simulink library "conventional_airplane_single_engine_lib"  (R2018b)
settings: Solver=VariableStepAuto  StartTime=0.0  StopTime=10.0  RelTol=1e-3
undefined symbols (not defined in the file or in its folder): airplane
libraries: actuators_lib x5, conventional_airplane_aerodynamics_lib x1, ground_lib x1, propulsion_lib x1, rigidBody_lib x1, flight_parameters_lib x1
settings Model: Creator=Ybeyer  LastModifiedBy=fabian
settings SFSimCC: SimUseLocalCustomCode=off
settings RTWCC: RTWUseLocalCustomCode=off
settings CodeAppCC: StateflowObjectComments=on

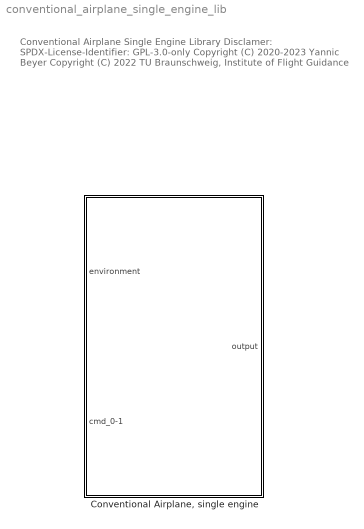
== system conventional_airplane_single_engine_lib ==
  note: Conventional Airplane Single Engine Library
      |
      | Disclamer:
      | SPDX-License-Identifier: GPL-3.0-only
      |
      | Copyright (C) 2020-2023 Yannic Beyer
      | Copyright (C) 2022 TU Braunschweig, Institute of Flight Guidance
  "Conventional Airplane, single engine" : Subsystem  mask{airplane=airplane}
      mask prompts: airplane "airplane struct"
      mask DialogControl DescGroupVar Prompt: Conventional Airplane, singe engine
      mask DialogControl DescTextVar Prompt: See conventionalAirplaneLoadParams for more information about the parameter struct.

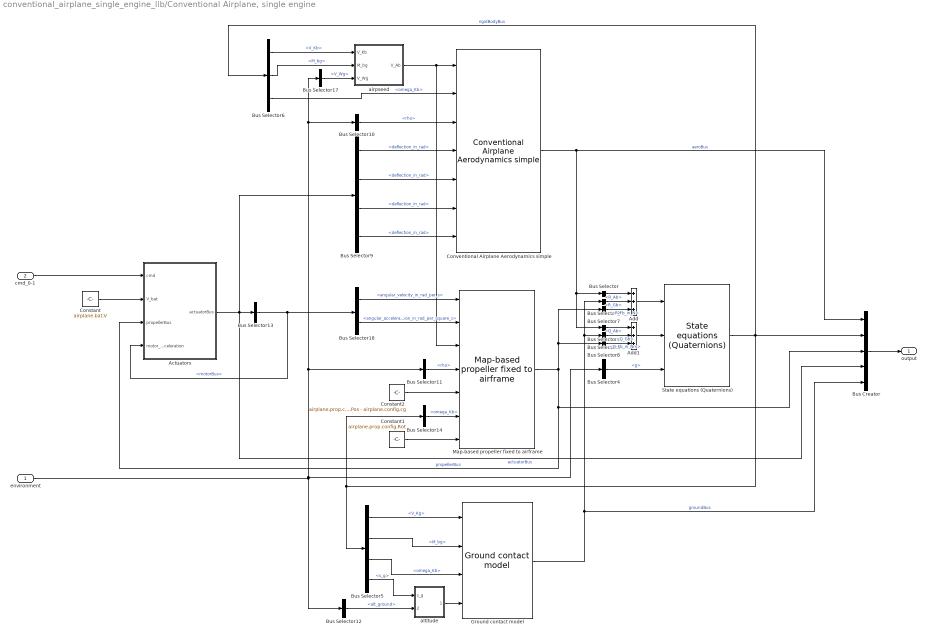
== system conventional_airplane_single_engine_lib/Conventional Airplane, single engine ==
  environment : Inport  OutDataTypeStr=Bus: envirBus
  cmd_0-1 : Inport  Port=2  OutDataTypeStr=Bus: cmdBus
  Actuators : Subsystem
  Add : Sum  Inputs=+++
  Add1 : Sum  Inputs=+++
  Bus Creator : BusCreator  Inputs=5
  Bus Selector : BusSelector  OutputSignals=R_Ab
  Bus Selector1 : BusSelector  OutputSignals=Q_Ab
  Bus Selector10 : BusSelector  OutputSignals=atmosphere.rho
  Bus Selector11 : BusSelector  OutputSignals=atmosphere.rho
  Bus Selector12 : BusSelector  OutputSignals=alt_ground
  Bus Selector13 : BusSelector  OutputSignals=motorBus
  Bus Selector14 : BusSelector  OutputSignals=omega_Kb
  Bus Selector17 : BusSelector  OutputSignals=wind.V_Wg
  Bus Selector18 : BusSelector  OutputSignals=angular_velocity_in_rad_per_s,angular_acceleration_in_rad_per_square_s
  Bus Selector2 : BusSelector  OutputSignals=forces_and_moments.R_Gb
  Bus Selector3 : BusSelector  OutputSignals=forces_and_moments.Q_Gb
  Bus Selector4 : BusSelector  OutputSignals=g
  Bus Selector5 : BusSelector  OutputSignals=V_Kg,M_bg,omega_Kb,s_g
  Bus Selector6 : BusSelector  OutputSignals=V_Kb,M_bg,omega_Kb
  Bus Selector7 : BusSelector  OutputSignals=R_Fb_in_N
  Bus Selector8 : BusSelector  OutputSignals=Q_Fb_in_Nm
  Bus Selector9 : BusSelector  OutputSignals=aileronsBus.deflection_in_rad,elevatorBus.deflection_in_rad,rudderBus.deflection_in_rad,htpTrimBus.deflection_in_rad
  Constant : Constant  Value=airplane.bat.V
  Constant1 : Constant  Value=airplane.prop.config.Rot
  Constant2 : Constant  Value=airplane.prop.config.Pos - airplane.config.cg
  Conventional Airplane Aerodynamics simple : conventional_airplane_aerodynamics_lib/Conventional Airplane Aerodynamics simple  aeroStruct=airplane.aero  xyz_cg_c=airplane.config.cg
      settings: SourceProductName=LADAC
  Ground contact model : ground_lib/Ground contact model  m=airplane.body.m  a_max=airplane.grnd.acc_max  xyz_c_hit=airplane.config.hitPoints  xyz_c_cg=airplane.config.cg  ground_softness_param=airplane.grnd.softness_parameter  k_h=airplane.grnd.spring_stiffness  k_dot_h=airplane.grnd.damping  mu=airplane.grnd.friction_coef  k_V=airplane.grnd.low_speed_friction_reduction_factor
      settings: SourceProductName=LADAC
  Map-based propeller fixed to airframe : propulsion_lib/Map-based propeller fixed to airframe  prop_map_fit=airplane.prop.map_fit  I_prop=airplane.prop.I  rotation_orientation=airplane.prop.dir
      settings: SourceProductName=LADAC
  State equations (Quaternions) : rigidBody_lib/State equations (Quaternions)  m=airplane.body.m  I=airplane.body.I  is_g_checked=on  g=10  omega_Kb_0=airplane.ic.omega_Kb  q_bg_0=airplane.ic.q_bg  V_Kb_0=airplane.ic.V_Kb  s_g_0=airplane.ic.s_Kg
      settings: SourceProductName=LADAC
  airpseed : Subsystem
  altitude : Subsystem
  output : Outport
  wires:
  Conventional Airplane Aerodynamics simple/1 -> Bus Selector1/1, Bus Selector/1, Bus Creator/1  "aeroBus"
  Bus Selector/1 -> Add/1  "<R_Ab>"
  Add/1 -> State equations (Quaternions)/1
  Add1/1 -> State equations (Quaternions)/2
  Bus Selector1/1 -> Add1/1  "<Q_Ab>"
  Bus Selector2/1 -> Add/2  "<R_Gb>"
  Ground contact model/1 -> Bus Creator/5, Bus Selector2/1, Bus Selector3/1  "groundBus"
  Bus Selector3/1 -> Add1/2  "<Q_Gb>"
  Bus Selector4/1 -> State equations (Quaternions)/3  "<g>"
  environment/1 -> Bus Selector11/1, Bus Selector17/1, Bus Selector10/1, Bus Selector4/1, Bus Selector12/1
  State equations (Quaternions)/1 -> Bus Selector6/1, Bus Creator/2, Bus Selector14/1, Bus Selector5/1  "rigidBodyBus"
  Bus Selector5/3 -> Ground contact model/3  "<omega_Kb>"
  Bus Selector5/2 -> Ground contact model/2  "<M_bg>"
  Bus Selector5/1 -> Ground contact model/1  "<V_Kg>"
  Bus Selector6/3 -> Conventional Airplane Aerodynamics simple/2  "<omega_Kb>"
  Bus Selector7/1 -> Add/3  "<R_Fb_in_N>"
  Map-based propeller fixed to airframe/1 -> Actuators/3(propellerBus), Bus Creator/3, Bus Selector8/1, Bus Selector7/1  "propellerBus"
  Bus Selector8/1 -> Add1/3  "<Q_Fb_in_Nm>"
  cmd_0-1/1 -> Actuators/1(cmd)
  Bus Selector9/1 -> Conventional Airplane Aerodynamics simple/4  "<deflection_in_rad>"
  Bus Selector9/2 -> Conventional Airplane Aerodynamics simple/5  "<deflection_in_rad>"
  Bus Selector9/3 -> Conventional Airplane Aerodynamics simple/6  "<deflection_in_rad>"
  Bus Selector9/4 -> Conventional Airplane Aerodynamics simple/7  "<deflection_in_rad>"
  Bus Selector10/1 -> Conventional Airplane Aerodynamics simple/3  "<rho>"
  Bus Selector11/1 -> Map-based propeller fixed to airframe/4  "<rho>"
  Bus Selector12/1 -> altitude/2(h_ground)  "<alt_ground>"
  altitude/1(alt_cg) -> Ground contact model/4
  Bus Selector14/1 -> Map-based propeller fixed to airframe/6  "<omega_Kb>"
  Bus Selector5/4 -> altitude/1(s_g)  "<s_g>"
  airpseed/1(V_Ab) -> Map-based propeller fixed to airframe/3, Conventional Airplane Aerodynamics simple/1
  Bus Selector6/1 -> airpseed/1(V_Kb)  "<V_Kb>"
  Bus Selector6/2 -> airpseed/2(M_bg)  "<M_bg>"
  Bus Selector17/1 -> airpseed/3(V_Wg)  "<V_Wg>"
  Bus Creator/1 -> output/1
  Constant1/1 -> Map-based propeller fixed to airframe/7
  Constant2/1 -> Map-based propeller fixed to airframe/5
  Bus Selector18/1 -> Map-based propeller fixed to airframe/1  "<angular_velocity_in_rad_per_s>"
  Bus Selector18/2 -> Map-based propeller fixed to airframe/2  "<angular_acceleration_in_rad_per_square_s>"
  Bus Selector13/1 -> Actuators/4(motor_acceleration), Bus Selector18/1  "<motorBus>"
  Constant/1 -> Actuators/2(V_bat)
  Actuators/1(actuatorBus) -> Bus Selector9/1, Bus Creator/4, Bus Selector13/1  "actuatorBus"

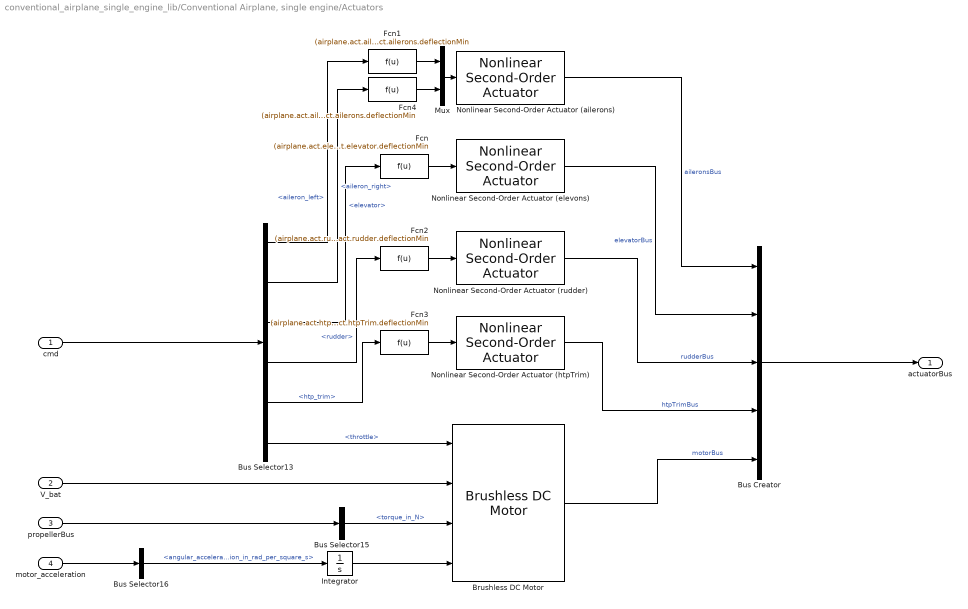
== system conventional_airplane_single_engine_lib/Conventional Airplane, single engine/Actuators ==
  cmd : Inport
  V_bat : Inport  Port=2
  propellerBus : Inport  Port=3
  motor_acceleration : Inport  Port=4
  Brushless DC Motor : actuators_lib/Brushless DC Motor  K_T=airplane.motor.KT  J_prop=airplane.prop.I  R_i=airplane.motor.R  IC_omega=0  omega_max=Inf  omega_min=0
      settings: SourceProductName=LADAC
  Bus Creator : BusCreator  Inputs=5
  Bus Selector13 : BusSelector  OutputSignals=aileron_left,aileron_right,elevator,rudder,htp_trim,throttle
  Bus Selector15 : BusSelector  OutputSignals=torque_in_N
  Bus Selector16 : BusSelector  OutputSignals=angular_acceleration_in_rad_per_square_s
  Fcn : Fcn  Expr=(airplane.act.elevator.deflectionMax - airplane.act.elevator.deflectionMin)*u + airplane.act.elevator.deflectionMin
  Fcn1 : Fcn  Expr=(airplane.act.ailerons.deflectionMax - airplane.act.ailerons.deflectionMin)*u + airplane.act.ailerons.deflectionMin
  Fcn2 : Fcn  Expr=(airplane.act.rudder.deflectionMax - airplane.act.rudder.deflectionMin)*u + airplane.act.rudder.deflectionMin
  Fcn3 : Fcn  Expr=(airplane.act.htpTrim.deflectionMax - airplane.act.htpTrim.deflectionMin)*u + airplane.act.htpTrim.deflectionMin
  Fcn4 : Fcn  Expr=(airplane.act.ailerons.deflectionMax - airplane.act.ailerons.deflectionMin)*u + airplane.act.ailerons.deflectionMin
  Integrator : Integrator  InitialCondition=airplane.ic.motor_speed  ContinuousStateAttributes='motor_speed'
  Mux : Mux  Inputs=2
  Nonlinear Second-Order Actuator (ailerons) : actuators_lib/Nonlinear Second-Order Actuator  omega=airplane.act.ailerons.naturalFrequency  d=airplane.act.ailerons.dampingRatio  A_max=airplane.act.ailerons.deflectionMax  A_min=airplane.act.ailerons.deflectionMin  dot_A_max=airplane.act.ailerons.deflectionRateMax  dot_A_min=-airplane.act.ailerons.deflectionRateMax  A_0=0  dot_A_0=0
      settings: SourceProductName=LADAC
  Nonlinear Second-Order Actuator (elevons) : actuators_lib/Nonlinear Second-Order Actuator  omega=airplane.act.elevator.naturalFrequency  d=airplane.act.elevator.dampingRatio  A_max=airplane.act.elevator.deflectionMax  A_min=airplane.act.elevator.deflectionMin  dot_A_max=airplane.act.elevator.deflectionRateMax  dot_A_min=-airplane.act.elevator.deflectionRateMax  A_0=0  dot_A_0=0
      settings: SourceProductName=LADAC
  Nonlinear Second-Order Actuator (htpTrim) : actuators_lib/Nonlinear Second-Order Actuator  omega=airplane.act.htpTrim.naturalFrequency  d=airplane.act.htpTrim.dampingRatio  A_max=airplane.act.htpTrim.deflectionMax  A_min=airplane.act.htpTrim.deflectionMin  dot_A_max=airplane.act.htpTrim.deflectionRateMax  dot_A_min=-airplane.act.htpTrim.deflectionRateMax  A_0=0  dot_A_0=0
      settings: SourceProductName=LADAC
  Nonlinear Second-Order Actuator (rudder) : actuators_lib/Nonlinear Second-Order Actuator  omega=airplane.act.rudder.naturalFrequency  d=airplane.act.rudder.dampingRatio  A_max=airplane.act.rudder.deflectionMax  A_min=airplane.act.rudder.deflectionMin  dot_A_max=airplane.act.rudder.deflectionRateMax  dot_A_min=-airplane.act.rudder.deflectionRateMax  A_0=0  dot_A_0=0
      settings: SourceProductName=LADAC
  actuatorBus : Outport
  wires:
  Bus Selector13/6 -> Brushless DC Motor/1  "<throttle>"
  Bus Selector16/1 -> Integrator/1  "<angular_acceleration_in_rad_per_square_s>"
  Bus Selector15/1 -> Brushless DC Motor/3  "<torque_in_N>"
  motor_acceleration/1 -> Bus Selector16/1
  Integrator/1 -> Brushless DC Motor/4
  Brushless DC Motor/1 -> Bus Creator/5  "motorBus"
  cmd/1 -> Bus Selector13/1
  V_bat/1 -> Brushless DC Motor/2
  propellerBus/1 -> Bus Selector15/1
  Bus Creator/1 -> actuatorBus/1
  Nonlinear Second-Order Actuator (rudder)/1 -> Bus Creator/3  "rudderBus"
  Nonlinear Second-Order Actuator (elevons)/1 -> Bus Creator/2  "elevatorBus"
  Nonlinear Second-Order Actuator (ailerons)/1 -> Bus Creator/1  "aileronsBus"
  Bus Selector13/1 -> Fcn1/1  "<aileron_left>"
  Bus Selector13/3 -> Fcn/1  "<elevator>"
  Bus Selector13/4 -> Fcn2/1  "<rudder>"
  Bus Selector13/2 -> Fcn4/1  "<aileron_right>"
  Bus Selector13/5 -> Fcn3/1  "<htp_trim>"
  Nonlinear Second-Order Actuator (htpTrim)/1 -> Bus Creator/4  "htpTrimBus"
  Fcn/1 -> Nonlinear Second-Order Actuator (elevons)/1
  Mux/1 -> Nonlinear Second-Order Actuator (ailerons)/1
  Fcn2/1 -> Nonlinear Second-Order Actuator (rudder)/1
  Fcn3/1 -> Nonlinear Second-Order Actuator (htpTrim)/1
  Fcn1/1 -> Mux/1
  Fcn4/1 -> Mux/2

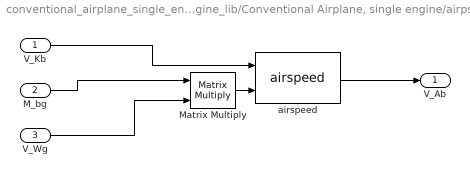
== system conventional_airplane_single_engine_lib/Conventional Airplane, single engine/airpseed ==
  V_Kb : Inport
  M_bg : Inport  Port=2
  V_Wg : Inport  Port=3
  Matrix Multiply : Product  Multiplication=Matrix(*)
  airspeed : flight_parameters_lib/airspeed
      settings: SourceProductName=LADAC
  V_Ab : Outport
  wires:
  V_Kb/1 -> airspeed/1
  Matrix Multiply/1 -> airspeed/2
  M_bg/1 -> Matrix Multiply/1
  airspeed/1 -> V_Ab/1
  V_Wg/1 -> Matrix Multiply/2

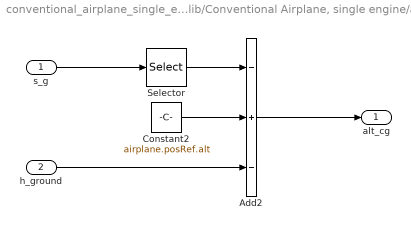
== system conventional_airplane_single_engine_lib/Conventional Airplane, single engine/altitude ==
  s_g : Inport
  h_ground : Inport  Port=2
  Add2 : Sum  Inputs=-+-
  Constant2 : Constant  Value=airplane.posRef.alt
  Selector : Selector  InputPortWidth=3  IndexOptions=Index vector (dialog)  Indices=3  OutputSizes=1
  alt_cg : Outport
  wires:
  s_g/1 -> Selector/1
  Constant2/1 -> Add2/2
  Add2/1 -> alt_cg/1
  Selector/1 -> Add2/1
  h_ground/1 -> Add2/3
